simulink model "OpenLoop"  (Simulink 10.2)
settings: Solver=ode4  StartTime=0.0  StopTime=TMax  FixedStep=DT  MaxStep=DT  RelTol=1e-3  EnableMultiTasking=on
settings Model: Creator=bjonkman  LastModifiedBy=aplatt
settings DataIOCC: LimitDataPoints=on  SaveOutput=off  SaveTime=off  SignalLoggingName=sigsOut
settings OptimizationCC: ExpressionDepthLimit=2147483647
settings DebuggingCC: SaveWithParameterizedLinksMsg=none  SignalResolutionControl=TryResolveAllWithWarning  MultiTaskDSMMsg=warning  MultiTaskCondExecSysMsg=none  StateNameClashWarn=warning
settings HardwareCC: TargetUnknown=on

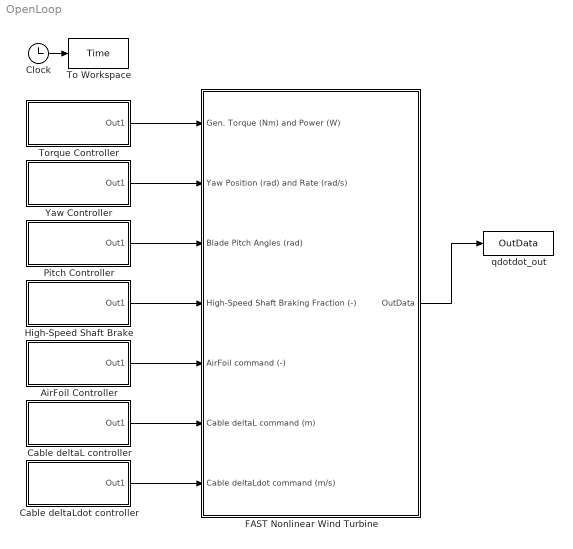
== system OpenLoop ==
  AirFoil Controller : Subsystem
  Cable deltaL controller : Subsystem
  Cable deltaLdot controller : Subsystem
  Clock : Clock
  FAST Nonlinear Wind Turbine : Subsystem  mask(FAST Nonlinear Wind Turbine){}
      mask help: This block contains the FAST S-Function.
      mask init:
      | clear FAST_SFunc
  High-Speed Shaft Brake : Subsystem
  Pitch Controller : Subsystem
  To Workspace : ToWorkspace  VariableName=Time  SampleTime=-1
  Torque Controller : Subsystem
  Yaw Controller : Subsystem
  qdotdot_out : ToWorkspace  VariableName=OutData  SampleTime=-1
  wires:
  Clock/1 -> To Workspace/1
  FAST Nonlinear Wind Turbine/1(OutData) -> qdotdot_out/1
  Torque Controller/1(Out1) -> FAST Nonlinear Wind Turbine/1(Gen. Torque (Nm) and Power (W))
  Yaw Controller/1(Out1) -> FAST Nonlinear Wind Turbine/2(Yaw Position (rad) and Rate (rad/s))
  Pitch Controller/1(Out1) -> FAST Nonlinear Wind Turbine/3(Blade Pitch Angles (rad))
  High-Speed Shaft Brake/1(Out1) -> FAST Nonlinear Wind Turbine/4(High-Speed Shaft Braking Fraction (-))
  AirFoil Controller/1(Out1) -> FAST Nonlinear Wind Turbine/5(AirFoil command (-))
  Cable deltaL controller/1(Out1) -> FAST Nonlinear Wind Turbine/6(Cable deltaL command (m))
  Cable deltaLdot controller/1(Out1) -> FAST Nonlinear Wind Turbine/7(Cable deltaLdot command (m/s))

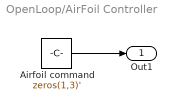
== system OpenLoop/AirFoil Controller ==
  Airfoil command : Constant  Value=zeros(1,3)'
  Out1 : Outport
  wires:
  Airfoil command/1 -> Out1/1

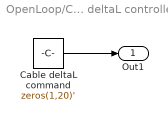
== system OpenLoop/Cable deltaL controller ==
  Cable deltaL command : Constant  Value=zeros(1,20)'
  Out1 : Outport
  wires:
  Cable deltaL command/1 -> Out1/1

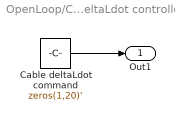
== system OpenLoop/Cable deltaLdot controller ==
  Cable deltaLdot command : Constant  Value=zeros(1,20)'
  Out1 : Outport
  wires:
  Cable deltaLdot command/1 -> Out1/1

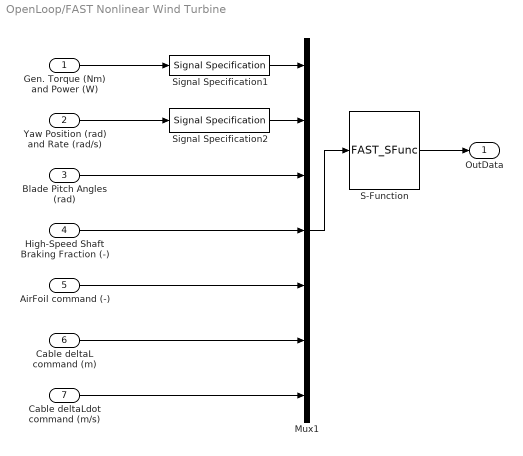
== system OpenLoop/FAST Nonlinear Wind Turbine ==
  Gen. Torque (Nm) and Power (W) : Inport
  Yaw Position (rad) and Rate (rad/s) : Inport  Port=2
  Blade Pitch Angles (rad) : Inport  Port=3
  High-Speed Shaft Braking Fraction (-) : Inport  Port=4
  AirFoil command (-) : Inport  Port=5
  Cable deltaL command (m) : Inport  Port=6
  Cable deltaLdot command (m/s) : Inport  Port=7
  Mux1 : Mux  Inputs=7
  S-Function : S-Function  FunctionName=FAST_SFunc  Parameters=FAST_InputFileName, TMax, 0  SFunctionDeploymentMode=off  EnableBusSupport=off
  Signal Specification1 : SignalSpecification  OutDataTypeStr=double  Dimensions=2
  Signal Specification2 : SignalSpecification  OutDataTypeStr=double  Dimensions=2
  OutData : Outport
  wires:
  Gen. Torque (Nm) and Power (W)/1 -> Signal Specification1/1
  S-Function/1 -> OutData/1
  Mux1/1 -> S-Function/1
  Blade Pitch Angles (rad)/1 -> Mux1/3
  Yaw Position (rad) and Rate (rad/s)/1 -> Signal Specification2/1
  Signal Specification1/1 -> Mux1/1
  Signal Specification2/1 -> Mux1/2
  High-Speed Shaft Braking Fraction (-)/1 -> Mux1/4
  AirFoil command (-)/1 -> Mux1/5
  Cable deltaL command (m)/1 -> Mux1/6
  Cable deltaLdot command (m/s)/1 -> Mux1/7

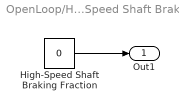
== system OpenLoop/High-Speed Shaft Brake ==
  High-Speed Shaft Braking Fraction : Constant  Value=0
  Out1 : Outport
  wires:
  High-Speed Shaft Braking Fraction/1 -> Out1/1

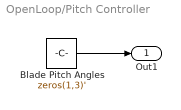
== system OpenLoop/Pitch Controller ==
  Blade Pitch Angles : Constant  Value=zeros(1,3)'
  Out1 : Outport
  wires:
  Blade Pitch Angles/1 -> Out1/1

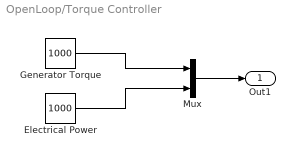
== system OpenLoop/Torque Controller ==
  Electrical Power : Constant  Value=1000
  Generator Torque : Constant  Value=1000
  Mux : Mux  Inputs=2
  Out1 : Outport
  wires:
  Mux/1 -> Out1/1
  Generator Torque/1 -> Mux/1
  Electrical Power/1 -> Mux/2

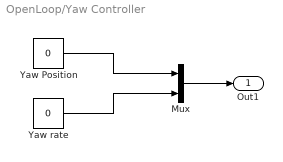
== system OpenLoop/Yaw Controller ==
  Mux : Mux  Inputs=2
  Yaw Position : Constant  Value=0
  Yaw rate : Constant  Value=0
  Out1 : Outport
  wires:
  Mux/1 -> Out1/1
  Yaw Position/1 -> Mux/1
  Yaw rate/1 -> Mux/2
